simulink model "softdrone_pid"  (R2023b)
settings: Solver=FixedStepAuto  StartTime=0.0  StopTime=Inf  FixedStep=0.001  RelTol=1e-3
values from neighbouring files (symbols this model uses):
  DEG2RAD = 0.0174533    [Init_control450.m]
  K_ROLL_AngleRate = 1.0    (= 1)    [Init_control450.m]
  Kd_PITCH_AngleRate = 0.003    [Init_control450.m]
  Kd_ROLL_AngleRate = 0.003    [Init_control450.m]
  Kd_YAW_AngleRate = 0.01    [Init_control450.m]
  Ki_PITCH_AngleRate = 0.002    [Init_control450.m]
  Ki_ROLL_AngleRate = 0.002    [Init_control450.m]
  Ki_YAW_AngleRate = 0.0    (= 0)    [Init_control450.m]
  Kp_ANGLE = 1.0    (= 1)    [Init_control450.m]
  Kp_ROLL_AngleRate = 0.122    [Init_control450.m]
  Kp_YAW_AngleRate = 1.0    (= 1)    [Init_control450.m]
  MAX_CONTROL_ANGLE_PITCH = 35    [Init_control450.m]
  MAX_CONTROL_ANGLE_RATE_PITCH = 350    [Init_control450.m]
  MAX_CONTROL_ANGLE_RATE_ROLL = 350    [Init_control450.m]
  MAX_CONTROL_ANGLE_RATE_YAW = 250    [Init_control450.m]
  MAX_CONTROL_ANGLE_ROLL = 35    [Init_control450.m]
  Saturation_I_RP_Max = 0.3    [Init_control450.m]
  Saturation_I_RP_Min = -0.3    [Init_control450.m]
  THR_HOVER = 0.609    [Init_control450.m]
  TIME_Constant = 0.1    [Init_control450.m]
undefined symbols (not defined in the file or in its folder): DiscIntNeverNeededParam
libraries: ros2lib x7, simulink x3
settings Model: SimulationMode=external  Creator=hang  LastModifiedBy=root
settings SolverCC: AlgebraicLoopSolver=TrustRegion  AutoInsertRateTranBlk=on  DecoupledContinuousIntegration=on  MinimalZcImpactIntegration=on
settings DataIOCC: ReturnWorkspaceOutputs=off
settings OptimizationCC: EnhancedBackFolding=on  PassReuseOutputArgsAs=Individual arguments  ZeroExternalMemoryAtStartup=off  ZeroInternalMemoryAtStartup=off  MaxStackSize=64  OptimizeBlockOrder=speed  DifferentSizesBufferReuse=on  OptimizationCustomize=off  EfficientTunableParamExpr=on
settings DebuggingCC: ParameterTunabilityLossMsg=error  UnconnectedInputMsg=warning  UnconnectedOutputMsg=warning  UnconnectedLineMsg=warning  ArithmeticOperatorsInVariantConditions=warning
settings HardwareCC: ProdBitPerLong=64  ProdHWDeviceType=AMD->x86-64 (Linux 64)
settings ModelReferenceCC: EnableRefExpFcnMdlSchedulingChecks=on
settings SFSimCC: SimUseLocalCustomCode=off  MATLABDynamicMemAlloc=off  CustomCodeUndefinedFunction=UseInterfaceOnly
settings RTWCC: Description=Embedded Coder  SystemTargetFile=ert.tlc  HardwareBoard=Robot Operating System 2 (ROS 2)  TLCOptions="-aInlineSetEventsForThisBaseRateFcn=TLC_FALSE -aSuppressMultiTaskScheduler=TLC_FALSE  -aRateBasedStepFcn=0"  GenCodeOnly=on  TemplateMakefile=ert_default_tmf  RTWUseLocalCustomCode=off  Toolchain=Colcon Tools  TargetLang=C++  DLArmComputeVersion=19.05
settings CodeAppCC: ForceParamTrailComments=on  IgnoreCustomStorageClasses=off  MaxIdLength=95  OperatorAnnotations=on  SimulinkDataObjDesc=on  SFDataObjDesc=on  InsertBlockDesc=on
settings ERTTargetCC: ExtMode=on  ExtModeMexArgs='127.0.0.1' 0 17725  RootIOFormat=Structure reference

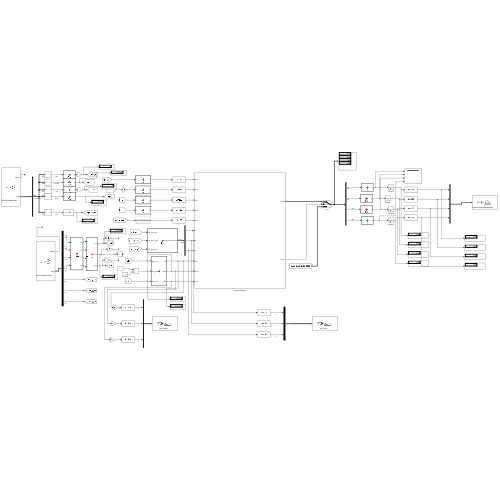
[thumbnail: Simulink's stored preview of the top-level diagram]
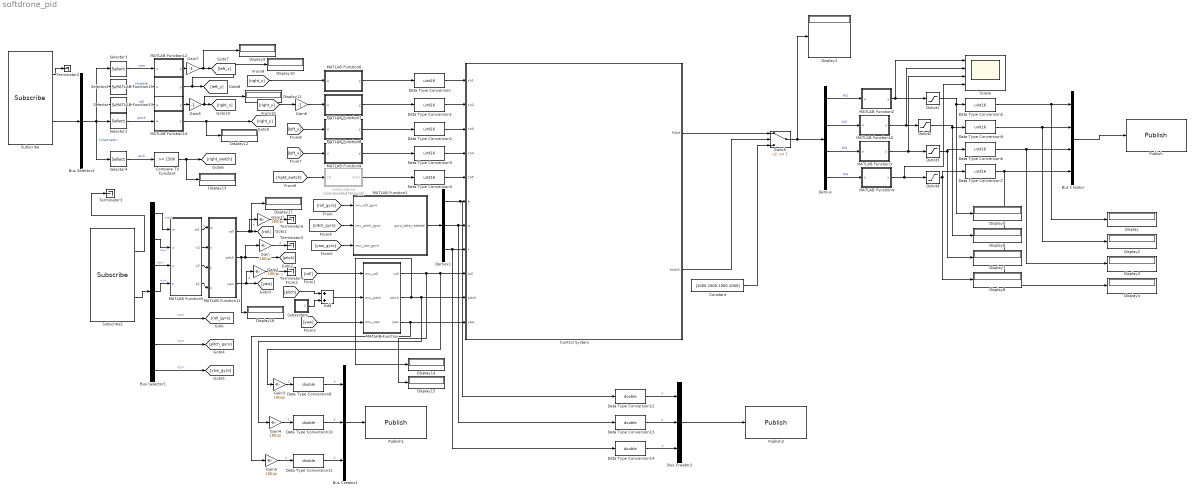
== system softdrone_pid ==
  Add : Sum
  Bus Creator : BusCreator  Inputs=4  OutDataTypeStr=Bus: SL_Bus_custom_msgs_WriteOnBoardPWM  NonVirtualBus=on
      settings: InheritFromInputs=off
  Bus Creator1 : BusCreator  Inputs=3  OutDataTypeStr=Bus: SL_Bus_geometry_msgs_Vector3  NonVirtualBus=on
  Bus Creator2 : BusCreator  Inputs=3  OutDataTypeStr=Bus: SL_Bus_geometry_msgs_Vector3  NonVirtualBus=on
  Bus Selector1 : BusSelector  OutputSignals=orientation.w,orientation.x,orientation.y,orientation.z,angular_velocity.x,angular_velocity.y,angular_velocity.z
  Bus Selector2 : BusSelector  OutputSignals=channels
  Compare To Constant : simulink/Logic and Bit Operations/Compare To Constant  relop=>=  const=1500  OutDataTypeStr=boolean
  Constant : Constant  Value=[1000,1000,1000,1000]
  Control System : Subsystem
  Data Type Conversion{,1..7,9} (9 alike) : DataTypeConversion  OutDataTypeStr=uint16  SaturateOnIntegerOverflow=off  RndMeth=Floor
  Data Type Conversion{8,10..14} (6 alike) : DataTypeConversion  OutDataTypeStr=double  SaturateOnIntegerOverflow=off  RndMeth=Floor
  Demux : Demux
  Demux1 : Demux  Outputs=3
  Display{,1..17} (18 alike) : Display
  Dshot{1..4} (4 alike) : Saturate  UpperLimit=2000  LowerLimit=1000
  Gain{,1..5} (6 alike) : Gain  Gain=180/pi
  Gain6 : Gain  Gain=-1
  Gain7 : Gain  Gain=-1
  Gain8 : Gain  Gain=-1
  MATLAB Function : MATLAB Function  TreatAsAtomicUnit=on
  MATLAB Function1 : MATLAB Function  TreatAsAtomicUnit=on
  MATLAB Function10 : MATLAB Function  TreatAsAtomicUnit=on
  MATLAB Function11 : MATLAB Function  TreatAsAtomicUnit=on
  MATLAB Function12 : MATLAB Function  TreatAsAtomicUnit=on
  MATLAB Function13 : MATLAB Function  TreatAsAtomicUnit=on
  MATLAB Function14 : MATLAB Function  TreatAsAtomicUnit=on
  MATLAB Function15 : MATLAB Function  TreatAsAtomicUnit=on
  MATLAB Function2 : MATLAB Function  TreatAsAtomicUnit=on
  MATLAB Function3 : MATLAB Function  TreatAsAtomicUnit=on
  MATLAB Function4 : MATLAB Function  TreatAsAtomicUnit=on
  MATLAB Function5 : MATLAB Function  TreatAsAtomicUnit=on
  MATLAB Function6 : MATLAB Function  TreatAsAtomicUnit=on
  MATLAB Function7 : MATLAB Function  TreatAsAtomicUnit=on
  MATLAB Function8 : MATLAB Function  TreatAsAtomicUnit=on
  MATLAB Function9 : MATLAB Function  TreatAsAtomicUnit=on
  Publish : ros2lib/Publish  topicSource=Select from ROS network  topic=/ecat/sn1966143/app3/write  messageType=custom_msgs/WriteOnBoardPWM  QOSHistory=Keep last  QOSDepth=1  QOSReliability=Best effort  QOSDurability=Volatile
  Publish1 : ros2lib/Publish  topicSource=Specify your own  topic=/imu_angle  messageType=geometry_msgs/Vector3  QOSHistory=Keep last  QOSDepth=1  QOSReliability=Reliable  QOSDurability=Volatile
  Publish2 : ros2lib/Publish  topicSource=Specify your own  topic=/imu_gyro  messageType=geometry_msgs/Vector3  QOSHistory=Keep all  QOSDepth=1  QOSReliability=Reliable  QOSDurability=Volatile
  Scope : Scope  NumInputPorts=4
  Selector : Selector  InputPortWidth=128  IndexOptions=Index vector (dialog)  Indices=1  OutputSizes=1
  Selector1 : Selector  InputPortWidth=128  IndexOptions=Index vector (dialog)  Indices=2  OutputSizes=1
  Selector2 : Selector  InputPortWidth=128  IndexOptions=Index vector (dialog)  Indices=3  OutputSizes=1
  Selector3 : Selector  InputPortWidth=128  IndexOptions=Index vector (dialog)  Indices=4  OutputSizes=1
  Selector4 : Selector  InputPortWidth=128  IndexOptions=Index vector (dialog)  Indices=5  OutputSizes=1
  Subscribe : ros2lib/Subscribe  topicSource=Select from ROS network  topic=/ecat/sn1966143/app1/read  messageType=custom_msgs/ReadSBUSRC  sampleTime=-1  QOSHistory=Keep last  QOSDepth=1  QOSReliability=Best effort  QOSDurability=Volatile
  Subscribe1 : ros2lib/Subscribe  topicSource=Select from ROS network  topic=/ecat/sn1966143/app2/read  messageType=sensor_msgs/Imu  sampleTime=-1  QOSHistory=Keep last  QOSDepth=1  QOSReliability=Best effort  QOSDurability=Volatile
  Subsystem : Subsystem
  Subsystem4 : Subsystem  Commented=through
  Switch : Switch  Threshold=1  SaturateOnIntegerOverflow=off  InputSameDT=off
  Terminator{2..6} (5 alike) : Terminator
  wires:
  Demux1/3 -> Data Type Conversion14/1, Control System/8(r)
  Demux1/1 -> Data Type Conversion12/1, Control System/6(p)
  MATLAB Function/2(pitch) -> Display14/1, Gain4/1, Control System/10(pitch)
  Demux1/2 -> Data Type Conversion13/1, Control System/7(q)
  Demux/4 -> MATLAB Function4/1(u)  "M4"
  Demux/3 -> MATLAB Function3/1(u)  "M3"
  Control System/1(PWM) -> Switch/1
  MATLAB Function1/1(gyro_data_rotated) -> Demux1/1
  MATLAB Function6/1(y) -> Data Type Conversion/1
  MATLAB Function9/1(y) -> Data Type Conversion3/1
  MATLAB Function8/1(y) -> Data Type Conversion2/1
  MATLAB Function7/1(y) -> Data Type Conversion1/1
  Subsystem4/1(Out1) -> Data Type Conversion4/1
  Control System/2(switch) -> Switch/2
  Data Type Conversion/1 -> Control System/1(ch1)
  Data Type Conversion1/1 -> Control System/2(ch2)
  Data Type Conversion2/1 -> Control System/3(ch3)
  Data Type Conversion3/1 -> Control System/4(ch4)
  Data Type Conversion4/1 -> Control System/5(ch5)
  Constant/1 -> Switch/3
  Switch/1 -> Display1/1, Demux/1
  Selector3/1 -> MATLAB Function12/1(u)  "yaw"
  Subscribe1/2 -> Bus Selector1/1
  Bus Creator/1 -> Publish/1
  MATLAB Function2/1(y) -> Scope/1, Dshot1/1
  MATLAB Function10/1(y) -> Scope/2, Dshot2/1
  MATLAB Function3/1(y) -> Scope/3, Dshot3/1
  MATLAB Function4/1(y) -> Scope/4, Dshot4/1
  Data Type Conversion5/1 -> Bus Creator/1, Display/1
  Data Type Conversion9/1 -> Bus Creator/2, Display2/1
  Data Type Conversion6/1 -> Bus Creator/3, Display3/1
  Data Type Conversion7/1 -> Bus Creator/4, Display4/1
  [roll_gyro] -> MATLAB Function1/1(imu_roll_gyro)
  [yaw] -> MATLAB Function/3(imu_yaw)
  [pitch_gyro] -> MATLAB Function1/2(imu_pitch_gyro)
  [yaw_gyro] -> MATLAB Function1/3(imu_yaw_gyro)
  [right_switch] -> Subsystem4/1(In1)
  [left_x] -> MATLAB Function9/1(u)
  [left_y] -> MATLAB Function8/1(u)
  Bus Selector1/7 -> [yaw_gyro]  "<z>"
  Bus Selector1/1 -> MATLAB Function5/1(w)  "<w>"
  Bus Selector1/4 -> MATLAB Function5/4(z)  "<z>"
  Subscribe/1 -> Terminator2/1
  Subscribe1/1 -> Terminator3/1
  Bus Selector1/2 -> MATLAB Function5/2(x)  "<x>"
  Bus Selector1/3 -> MATLAB Function5/3(y)  "<y>"
  MATLAB Function5/1(w2) -> MATLAB Function11/1(w)  "y"
  MATLAB Function5/2(x2) -> MATLAB Function11/2(x)
  MATLAB Function5/3(y2) -> MATLAB Function11/3(y)
  MATLAB Function5/4(z2) -> MATLAB Function11/4(z)
  Demux/1 -> MATLAB Function2/1(u)  "M1"
  Demux/2 -> MATLAB Function10/1(u)  "M2"
  MATLAB Function11/2(pitch) -> [pitch], Gain/1, Display16/1
  MATLAB Function11/3(yaw) -> Gain2/1, [yaw]  "z"
  MATLAB Function11/1(roll) -> Gain1/1, Display17/1, [roll]  "x"
  Bus Creator1/1 -> Publish1/1
  Data Type Conversion8/1 -> Bus Creator1/1  "x"
  Data Type Conversion10/1 -> Bus Creator1/2  "y"
  Data Type Conversion11/1 -> Bus Creator1/3  "z"
  Bus Creator2/1 -> Publish2/1
  Data Type Conversion12/1 -> Bus Creator2/1  "x"
  Data Type Conversion14/1 -> Bus Creator2/3  "z"
  Data Type Conversion13/1 -> Bus Creator2/2  "y"
  Bus Selector1/5 -> [roll_gyro]  "<x>"
  Bus Selector1/6 -> [pitch_gyro]  "<y>"
  Dshot2/1 -> Display6/1, Data Type Conversion9/1
  Dshot1/1 -> Display5/1, Data Type Conversion5/1
  Dshot3/1 -> Data Type Conversion6/1, Display7/1
  Dshot4/1 -> Display8/1, Data Type Conversion7/1
  MATLAB Function/3(yaw) -> Control System/11(yaw), Gain5/1
  Gain3/1 -> Data Type Conversion8/1  "z"
  Gain4/1 -> Data Type Conversion10/1  "z"
  Gain5/1 -> Data Type Conversion11/1  "z"
  Gain2/1 -> Terminator4/1  "z"
  Gain/1 -> Terminator5/1  "y"
  Gain1/1 -> Terminator6/1  "x"
  [right_y] -> Gain6/1
  [right_x] -> MATLAB Function6/1(u)
  Gain6/1 -> MATLAB Function7/1(u)
  Subscribe/2 -> Bus Selector2/1
  Bus Selector2/1 -> Selector4/1, Selector1/1, Selector3/1, Selector2/1, Selector/1  "<channels>"
  Selector/1 -> MATLAB Function13/1(u)  "roll"
  Selector1/1 -> MATLAB Function14/1(u)  "pitch"
  Selector2/1 -> MATLAB Function15/1(u)  "throttle"
  Selector4/1 -> Compare To Constant/1  "arm"
  MATLAB Function14/1(y) -> Display12/1, [right_y]
  MATLAB Function15/1(y) -> Display10/1, [left_y]
  Compare To Constant/1 -> Display13/1, [right_switch]
  MATLAB Function12/1(y) -> Gain7/1
  Gain7/1 -> Display9/1, [left_x]
  MATLAB Function13/1(y) -> Gain8/1
  Gain8/1 -> Display11/1, [right_x]
  MATLAB Function/1(roll) -> Display15/1, Gain3/1, Control System/9(roll)
  [roll] -> MATLAB Function/1(imu_roll)
  [pitch] -> Add/1
  Add/1 -> MATLAB Function/2(imu_pitch)
  Subsystem/1(Out1) -> Add/2

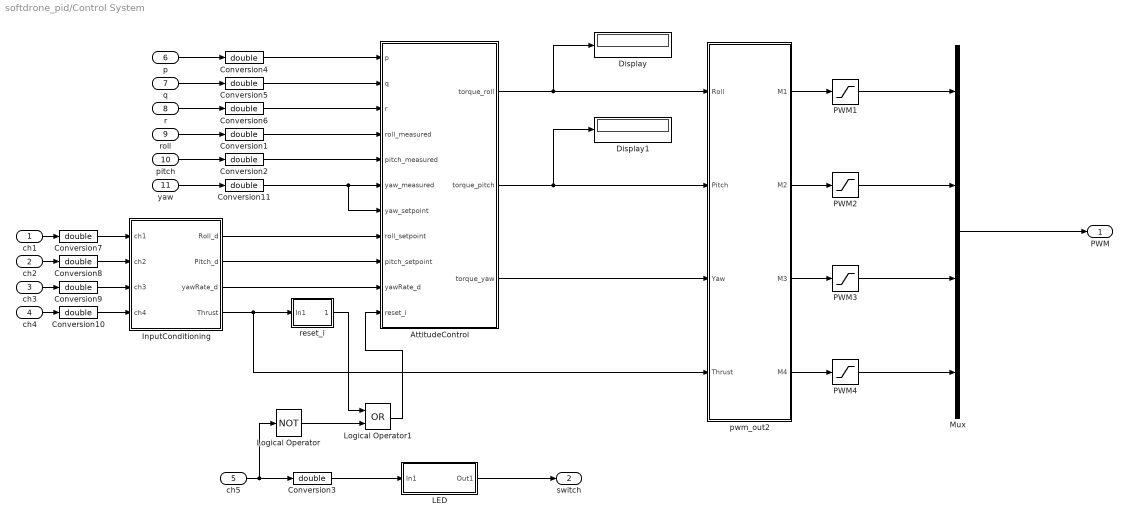
== system softdrone_pid/Control System ==
  ch1 : Inport  OutDataTypeStr=uint16  PortDimensions=1
  ch2 : Inport  Port=2  OutDataTypeStr=uint16  PortDimensions=1
  ch3 : Inport  Port=3  OutDataTypeStr=uint16  PortDimensions=1
  ch4 : Inport  Port=4  OutDataTypeStr=uint16  PortDimensions=1
  ch5 : Inport  Port=5  OutDataTypeStr=uint16  PortDimensions=1  Interpolate=off
  p : Inport  Port=6  PortDimensions=1
  q : Inport  Port=7  PortDimensions=1
  r : Inport  Port=8  PortDimensions=1
  roll : Inport  Port=9  PortDimensions=1
  pitch : Inport  Port=10  PortDimensions=1
  yaw : Inport  Port=11  PortDimensions=1
  AttitudeControl : Subsystem
  Conversion{1..11} (11 alike) : DataTypeConversion  OutDataTypeStr=double  SaturateOnIntegerOverflow=off  RndMeth=Floor
  Display : Display
  Display1 : Display
  InputConditioning : Subsystem
  "LED " : Subsystem
  Logical Operator : Logic  Operator=NOT  AllPortsSameDT=off  OutDataTypeStr=boolean
  Logical Operator1 : Logic  Operator=OR  AllPortsSameDT=off  OutDataTypeStr=boolean
  Mux : Mux
  PWM{1..4} (4 alike) : Saturate  UpperLimit=2000  LowerLimit=1200
  pwm_out2 : MATLAB Function  SystemSampleTime=0.004
  reset_i : Subsystem
  PWM : Outport  VectorParamsAs1DForOutWhenUnconnected=off
  switch : Outport  Port=2  PortDimensions=1  VectorParamsAs1DForOutWhenUnconnected=off
  wires:
  AttitudeControl/2(torque_pitch) -> Display1/1, pwm_out2/2(Pitch)
  AttitudeControl/3(torque_yaw) -> pwm_out2/3(Yaw)
  reset_i/1(Out1) -> Logical Operator1/1
  p/1 -> Conversion4/1
  q/1 -> Conversion5/1
  r/1 -> Conversion6/1
  pitch/1 -> Conversion2/1
  roll/1 -> Conversion1/1
  "LED "/1(Out1) -> switch/1
  ch5/1 -> Logical Operator/1, Conversion3/1
  Conversion3/1 -> "LED "/1(In1)
  ch3/1 -> Conversion9/1
  ch4/1 -> Conversion10/1
  Conversion10/1 -> InputConditioning/4(ch4)
  Conversion9/1 -> InputConditioning/3(ch3)
  ch1/1 -> Conversion7/1
  ch2/1 -> Conversion8/1
  InputConditioning/3(yawRate_d) -> AttitudeControl/10(yawRate_d)
  InputConditioning/4(Thrust) -> pwm_out2/4(Thrust), reset_i/1(In1)
  Conversion7/1 -> InputConditioning/1("ch1 ")
  Conversion8/1 -> InputConditioning/2(ch2)
  yaw/1 -> Conversion11/1
  Conversion6/1 -> AttitudeControl/3(r)
  Conversion5/1 -> AttitudeControl/2(q)
  Conversion4/1 -> AttitudeControl/1(p)
  Conversion11/1 -> AttitudeControl/6(yaw_measured), AttitudeControl/7(yaw_setpoint)
  Conversion2/1 -> AttitudeControl/5(pitch_measured)
  Conversion1/1 -> AttitudeControl/4(roll_measured)
  InputConditioning/2(Pitch_d) -> AttitudeControl/9(pitch_setpoint)
  InputConditioning/1(Roll_d) -> AttitudeControl/8(roll_setpoint)
  AttitudeControl/1(torque_roll) -> Display/1, pwm_out2/1(Roll)
  pwm_out2/4(M4) -> PWM4/1
  pwm_out2/3(M3) -> PWM3/1
  pwm_out2/1(M1) -> PWM1/1
  pwm_out2/2(M2) -> PWM2/1
  Mux/1 -> PWM/1
  PWM1/1 -> Mux/1
  PWM2/1 -> Mux/2
  PWM3/1 -> Mux/3
  PWM4/1 -> Mux/4
  Logical Operator/1 -> Logical Operator1/2
  Logical Operator1/1 -> AttitudeControl/11(reset_i)

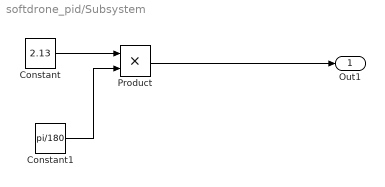
== system softdrone_pid/Subsystem ==
  Constant : Constant  Value=2.13
  Constant1 : Constant  Value=pi/180
  Product : Product
  Out1 : Outport
  wires:
  Constant/1 -> Product/1
  Constant1/1 -> Product/2
  Product/1 -> Out1/1

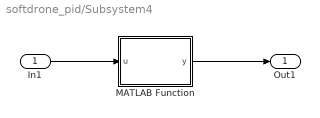
== system softdrone_pid/Subsystem4 ==
  In1 : Inport
  MATLAB Function : MATLAB Function  TreatAsAtomicUnit=on
  Out1 : Outport
  wires:
  In1/1 -> MATLAB Function/1(u)
  MATLAB Function/1(y) -> Out1/1

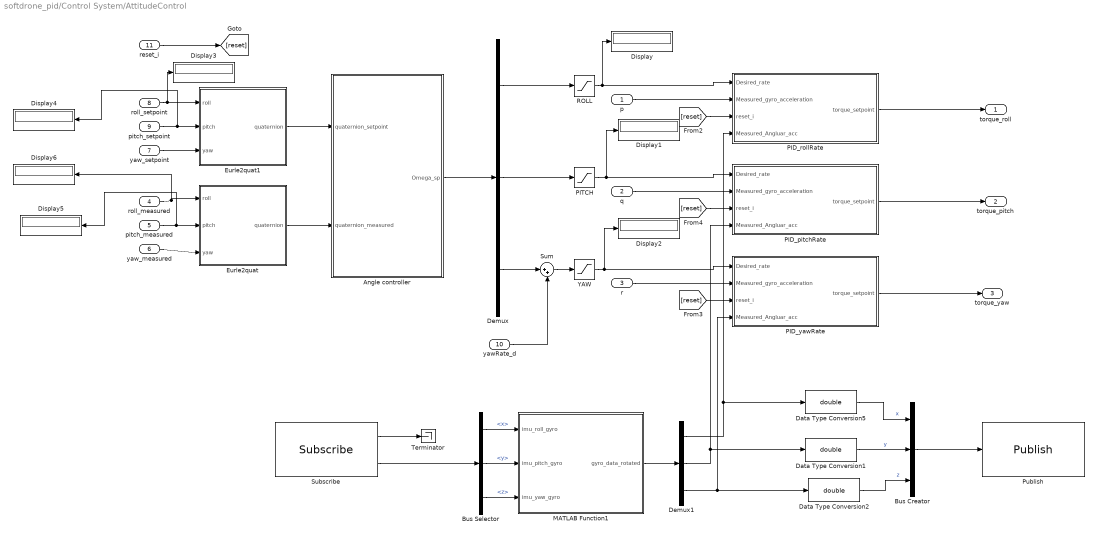
== system softdrone_pid/Control System/AttitudeControl ==
  p : Inport
  q : Inport  Port=2
  r : Inport  Port=3
  roll_measured : Inport  Port=4
  pitch_measured : Inport  Port=5
  yaw_measured : Inport  Port=6
  yaw_setpoint : Inport  Port=7
  roll_setpoint : Inport  Port=8
  pitch_setpoint : Inport  Port=9
  yawRate_d : Inport  Port=10
  reset_i : Inport  Port=11
  Angle controller : Subsystem
  Bus Creator : BusCreator  Inputs=3  OutDataTypeStr=Bus: SL_Bus_geometry_msgs_Vector3  NonVirtualBus=on
  Bus Selector : BusSelector  OutputSignals=x,y,z
  Data Type Conversion1 : DataTypeConversion  OutDataTypeStr=double  SaturateOnIntegerOverflow=off  RndMeth=Floor
  Data Type Conversion2 : DataTypeConversion  OutDataTypeStr=double  SaturateOnIntegerOverflow=off  RndMeth=Floor
  Data Type Conversion5 : DataTypeConversion  OutDataTypeStr=double  SaturateOnIntegerOverflow=off  RndMeth=Floor
  Demux : Demux  Outputs=3
  Demux1 : Demux  Outputs=3
  Display{,1..6} (7 alike) : Display
  Eurle2quat : MATLAB Function  TreatAsAtomicUnit=on
  Eurle2quat1 : MATLAB Function  TreatAsAtomicUnit=on
  MATLAB Function1 : MATLAB Function  TreatAsAtomicUnit=on
  PID_pitchRate : Subsystem
  PID_rollRate : Subsystem
  PID_yawRate : Subsystem
  PITCH : Saturate  UpperLimit=MAX_CONTROL_ANGLE_RATE_PITCH  LowerLimit=-MAX_CONTROL_ANGLE_RATE_PITCH
  Publish : ros2lib/Publish  topicSource=Specify your own  topic=/gyro_rotated  messageType=geometry_msgs/Vector3  QOSHistory=Keep last  QOSDepth=1  QOSReliability=Best effort  QOSDurability=Volatile
  ROLL : Saturate  UpperLimit=MAX_CONTROL_ANGLE_RATE_ROLL  LowerLimit=-MAX_CONTROL_ANGLE_RATE_ROLL
  Subscribe : ros2lib/Subscribe  topicSource=Select from ROS network  topic=/filtered_angular_acceleration  messageType=geometry_msgs/Vector3  sampleTime=-1  QOSHistory=Keep last  QOSDepth=1  QOSReliability=Reliable  QOSDurability=Volatile
  Sum : Sum  Inputs=|++
  Terminator : Terminator
  YAW : Saturate  UpperLimit=MAX_CONTROL_ANGLE_RATE_YAW  LowerLimit=-MAX_CONTROL_ANGLE_RATE_YAW
  torque_roll : Outport  VectorParamsAs1DForOutWhenUnconnected=off
  torque_pitch : Outport  Port=2  VectorParamsAs1DForOutWhenUnconnected=off
  torque_yaw : Outport  Port=3  VectorParamsAs1DForOutWhenUnconnected=off
  wires:
  p/1 -> PID_rollRate/2(Measured_gyro_acceleration)
  reset_i/1 -> [reset]
  [reset] -> PID_rollRate/3(reset_i)
  PID_rollRate/1(torque_setpoint) -> torque_roll/1
  [reset] -> PID_pitchRate/3(reset_i)
  PID_pitchRate/1(torque_setpoint) -> torque_pitch/1
  q/1 -> PID_pitchRate/2(Measured_gyro_acceleration)
  [reset] -> PID_yawRate/3(reset_i)
  PID_yawRate/1(torque_setpoint) -> torque_yaw/1
  r/1 -> PID_yawRate/2(Measured_gyro_acceleration)
  Eurle2quat/1(quaternion) -> Angle controller/2(quaternion_measured)
  roll_measured/1 -> Display6/1, Eurle2quat/1(roll)
  pitch_measured/1 -> Display5/1, Eurle2quat/2(pitch)
  yaw_measured/1 -> Eurle2quat/3(yaw)
  Eurle2quat1/1(quaternion) -> Angle controller/1(quaternion_setpoint)
  pitch_setpoint/1 -> Display4/1, Eurle2quat1/2(pitch)
  roll_setpoint/1 -> Display3/1, Eurle2quat1/1(roll)
  yaw_setpoint/1 -> Eurle2quat1/3(yaw)
  Demux/1 -> ROLL/1
  Demux/2 -> PITCH/1
  Angle controller/1(Omega_sp) -> Demux/1
  Demux/3 -> Sum/1
  Sum/1 -> YAW/1
  yawRate_d/1 -> Sum/2
  ROLL/1 -> Display/1, PID_rollRate/1(Desired_rate)
  PITCH/1 -> Display1/1, PID_pitchRate/1(Desired_rate)
  YAW/1 -> Display2/1, PID_yawRate/1(Desired_rate)
  Subscribe/1 -> Terminator/1
  Subscribe/2 -> Bus Selector/1
  Bus Selector/1 -> MATLAB Function1/1(imu_roll_gyro)  "<x>"
  Bus Selector/2 -> MATLAB Function1/2(imu_pitch_gyro)  "<y>"
  Bus Selector/3 -> MATLAB Function1/3(imu_yaw_gyro)  "<z>"
  MATLAB Function1/1(gyro_data_rotated) -> Demux1/1
  Demux1/1 -> Data Type Conversion5/1, PID_rollRate/4(Measured_Angluar_acc)
  Demux1/3 -> Data Type Conversion2/1, PID_yawRate/4(Measured_Angluar_acc)
  Demux1/2 -> Data Type Conversion1/1, PID_pitchRate/4(Measured_Angluar_acc)
  Data Type Conversion5/1 -> Bus Creator/1  "x"
  Data Type Conversion1/1 -> Bus Creator/2  "y"
  Data Type Conversion2/1 -> Bus Creator/3  "z"
  Bus Creator/1 -> Publish/1

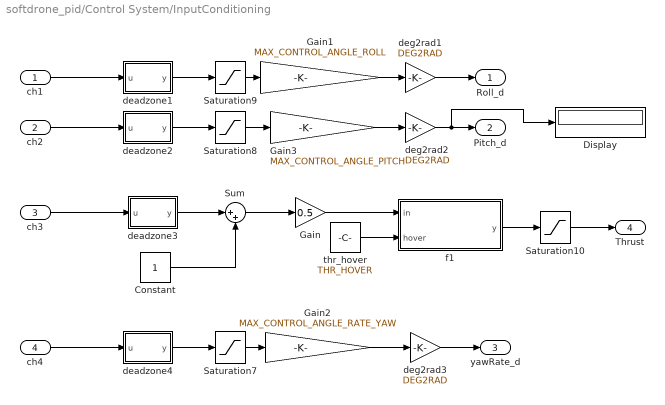
== system softdrone_pid/Control System/InputConditioning ==
  "ch1 " : Inport
  ch2 : Inport  Port=2
  ch3 : Inport  Port=3
  ch4 : Inport  Port=4
  Constant : Constant
  Display : Display
  Gain : Gain  Gain=0.5
  Gain1 : Gain  Gain=MAX_CONTROL_ANGLE_ROLL  OutDataTypeStr=Inherit: Inherit via back propagation
  Gain2 : Gain  Gain=MAX_CONTROL_ANGLE_RATE_YAW
  Gain3 : Gain  Gain=MAX_CONTROL_ANGLE_PITCH  OutDataTypeStr=Inherit: Inherit via back propagation
  Saturation10 : Saturate  UpperLimit=1  LowerLimit=0
  Saturation7 : Saturate  UpperLimit=1  LowerLimit=-1
  Saturation8 : Saturate  UpperLimit=1  LowerLimit=-1
  Saturation9 : Saturate  UpperLimit=1  LowerLimit=-1
  Sum : Sum  Inputs=|++
  deadzone1 : MATLAB Function  TreatAsAtomicUnit=on
  deadzone2 : MATLAB Function  TreatAsAtomicUnit=on
  deadzone3 : MATLAB Function  TreatAsAtomicUnit=on
  deadzone4 : MATLAB Function  TreatAsAtomicUnit=on
  deg2rad1 : Gain  Gain=DEG2RAD
  deg2rad2 : Gain  Gain=DEG2RAD
  deg2rad3 : Gain  Gain=DEG2RAD
  f1 : MATLAB Function  TreatAsAtomicUnit=on
  "thr_hover " : Constant  Value=THR_HOVER
  Roll_d : Outport  VectorParamsAs1DForOutWhenUnconnected=off
  Pitch_d : Outport  Port=2  VectorParamsAs1DForOutWhenUnconnected=off
  yawRate_d : Outport  Port=3  VectorParamsAs1DForOutWhenUnconnected=off
  Thrust : Outport  Port=4  VectorParamsAs1DForOutWhenUnconnected=off
  wires:
  deadzone3/1(y) -> Sum/1
  ch3/1 -> deadzone3/1(u)
  deadzone2/1(y) -> Saturation8/1
  Saturation10/1 -> Thrust/1
  deadzone1/1(y) -> Saturation9/1
  "ch1 "/1 -> deadzone1/1(u)
  ch2/1 -> deadzone2/1(u)
  Saturation9/1 -> Gain1/1
  Saturation8/1 -> Gain3/1
  Gain3/1 -> deg2rad2/1
  Constant/1 -> Sum/2
  Sum/1 -> Gain/1
  Gain1/1 -> deg2rad1/1
  deg2rad1/1 -> Roll_d/1
  deg2rad2/1 -> Display/1, Pitch_d/1
  Saturation7/1 -> Gain2/1
  deadzone4/1(y) -> Saturation7/1
  ch4/1 -> deadzone4/1(u)
  Gain2/1 -> deg2rad3/1
  deg2rad3/1 -> yawRate_d/1
  "thr_hover "/1 -> f1/2(hover)
  Gain/1 -> f1/1(in)
  f1/1(y) -> Saturation10/1

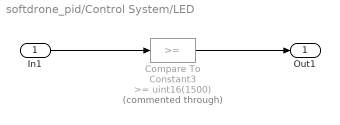
== system softdrone_pid/Control System/LED  ==
  In1 : Inport
  Compare To Constant3 : simulink/Logic and Bit Operations/Compare To Constant  Commented=through  relop=>=  const=uint16(1500)  OutDataTypeStr=boolean
  Out1 : Outport  VectorParamsAs1DForOutWhenUnconnected=off
  wires:
  Compare To Constant3/1 -> Out1/1
  In1/1 -> Compare To Constant3/1

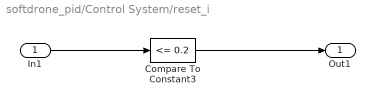
== system softdrone_pid/Control System/reset_i ==
  In1 : Inport
  Compare To Constant3 : simulink/Logic and Bit Operations/Compare To Constant  relop=<=  const=0.2  OutDataTypeStr=boolean
  Out1 : Outport  VectorParamsAs1DForOutWhenUnconnected=off
  wires:
  In1/1 -> Compare To Constant3/1
  Compare To Constant3/1 -> Out1/1

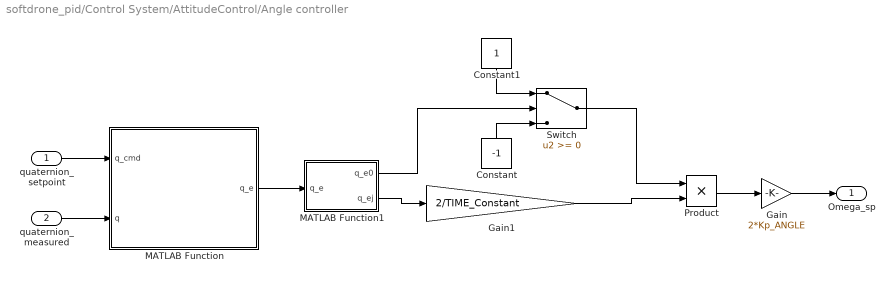
== system softdrone_pid/Control System/AttitudeControl/Angle controller ==
  quaternion_setpoint : Inport
  quaternion_measured : Inport  Port=2
  Constant : Constant  Value=-1
  Constant1 : Constant
  Gain : Gain  Gain=2*Kp_ANGLE
  Gain1 : Gain  Gain=2/TIME_Constant
  MATLAB Function : MATLAB Function  TreatAsAtomicUnit=on
  MATLAB Function1 : MATLAB Function  TreatAsAtomicUnit=on
  Product : Product
  Switch : Switch  SaturateOnIntegerOverflow=off  InputSameDT=off
  Omega_sp : Outport
  wires:
  quaternion_setpoint/1 -> MATLAB Function/1(q_cmd)
  quaternion_measured/1 -> MATLAB Function/2(q)
  Gain/1 -> Omega_sp/1
  Product/1 -> Gain/1
  MATLAB Function/1(q_e) -> MATLAB Function1/1(q_e)
  Gain1/1 -> Product/2
  MATLAB Function1/2(q_ej) -> Gain1/1
  MATLAB Function1/1(q_e0) -> Switch/2
  Switch/1 -> Product/1
  Constant/1 -> Switch/3
  Constant1/1 -> Switch/1

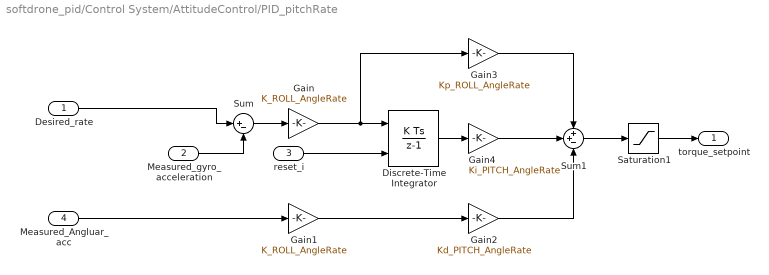
== system softdrone_pid/Control System/AttitudeControl/PID_pitchRate ==
  Desired_rate : Inport
  Measured_gyro_acceleration : Inport  Port=2
  reset_i : Inport  Port=3
  Measured_Angluar_acc : Inport  Port=4
  Discrete-Time Integrator : DiscreteIntegrator  ExternalReset=level  SampleTime=-1  LimitOutput=on  UpperSaturationLimit=Saturation_I_RP_Max  LowerSaturationLimit=Saturation_I_RP_Min  ICPrevOutput=DiscIntNeverNeededParam  ICPrevScaledInput=DiscIntNeverNeededParam
  Gain : Gain  Gain=K_ROLL_AngleRate
  Gain1 : Gain  Gain=K_ROLL_AngleRate
  Gain2 : Gain  Gain=Kd_PITCH_AngleRate
  Gain3 : Gain  Gain=Kp_ROLL_AngleRate
  Gain4 : Gain  Gain=Ki_PITCH_AngleRate
  Saturation1 : Saturate  UpperLimit=1  LowerLimit=-1
  Sum : Sum  Inputs=|+-
  Sum1 : Sum  Inputs=++-
  torque_setpoint : Outport
  wires:
  Gain2/1 -> Sum1/3
  Gain4/1 -> Sum1/2
  Gain3/1 -> Sum1/1
  Gain/1 -> Discrete-Time Integrator/1, Gain3/1
  Sum1/1 -> Saturation1/1
  Saturation1/1 -> torque_setpoint/1
  Discrete-Time Integrator/1 -> Gain4/1
  reset_i/1 -> Discrete-Time Integrator/2
  Gain1/1 -> Gain2/1
  Desired_rate/1 -> Sum/1
  Sum/1 -> Gain/1
  Measured_gyro_acceleration/1 -> Sum/2
  Measured_Angluar_acc/1 -> Gain1/1

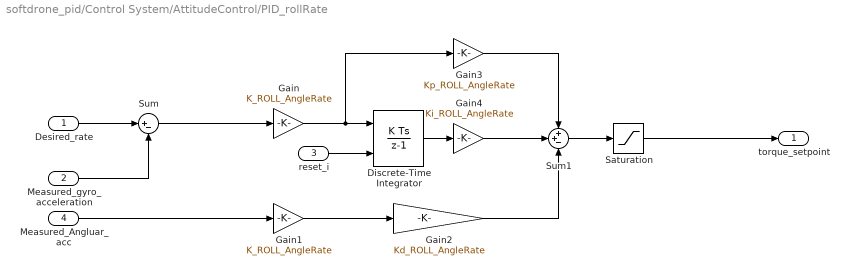
== system softdrone_pid/Control System/AttitudeControl/PID_rollRate ==
  Desired_rate : Inport
  Measured_gyro_acceleration : Inport  Port=2
  reset_i : Inport  Port=3
  Measured_Angluar_acc : Inport  Port=4
  Discrete-Time Integrator : DiscreteIntegrator  ExternalReset=level  SampleTime=-1  LimitOutput=on  UpperSaturationLimit=Saturation_I_RP_Max  LowerSaturationLimit=Saturation_I_RP_Min  ICPrevOutput=DiscIntNeverNeededParam  ICPrevScaledInput=DiscIntNeverNeededParam
  Gain : Gain  Gain=K_ROLL_AngleRate
  Gain1 : Gain  Gain=K_ROLL_AngleRate
  Gain2 : Gain  Gain=Kd_ROLL_AngleRate
  Gain3 : Gain  Gain=Kp_ROLL_AngleRate
  Gain4 : Gain  Gain=Ki_ROLL_AngleRate
  Saturation : Saturate  UpperLimit=1  LowerLimit=-1
  Sum : Sum  Inputs=|+-
  Sum1 : Sum  Inputs=++-
  torque_setpoint : Outport
  wires:
  Gain2/1 -> Sum1/3
  Gain4/1 -> Sum1/2
  Gain3/1 -> Sum1/1
  Gain/1 -> Discrete-Time Integrator/1, Gain3/1
  Sum1/1 -> Saturation/1
  Discrete-Time Integrator/1 -> Gain4/1
  reset_i/1 -> Discrete-Time Integrator/2
  Gain1/1 -> Gain2/1
  Desired_rate/1 -> Sum/1
  Measured_gyro_acceleration/1 -> Sum/2
  Sum/1 -> Gain/1
  Measured_Angluar_acc/1 -> Gain1/1
  Saturation/1 -> torque_setpoint/1

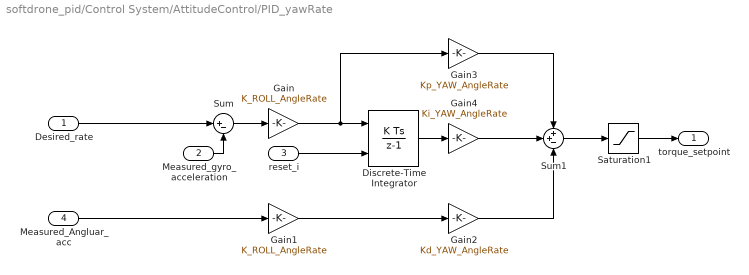
== system softdrone_pid/Control System/AttitudeControl/PID_yawRate ==
  Desired_rate : Inport
  Measured_gyro_acceleration : Inport  Port=2
  reset_i : Inport  Port=3
  Measured_Angluar_acc : Inport  Port=4
  Discrete-Time Integrator : DiscreteIntegrator  ExternalReset=level  SampleTime=-1  LimitOutput=on  UpperSaturationLimit=Saturation_I_RP_Max  LowerSaturationLimit=Saturation_I_RP_Min  ICPrevOutput=DiscIntNeverNeededParam  ICPrevScaledInput=DiscIntNeverNeededParam
  Gain : Gain  Gain=K_ROLL_AngleRate
  Gain1 : Gain  Gain=K_ROLL_AngleRate
  Gain2 : Gain  Gain=Kd_YAW_AngleRate
  Gain3 : Gain  Gain=Kp_YAW_AngleRate
  Gain4 : Gain  Gain=Ki_YAW_AngleRate
  Saturation1 : Saturate  UpperLimit=1  LowerLimit=-1
  Sum : Sum  Inputs=|+-
  Sum1 : Sum  Inputs=++-
  torque_setpoint : Outport
  wires:
  Gain2/1 -> Sum1/3
  Gain4/1 -> Sum1/2
  Gain3/1 -> Sum1/1
  Gain/1 -> Discrete-Time Integrator/1, Gain3/1
  Sum1/1 -> Saturation1/1
  Saturation1/1 -> torque_setpoint/1
  Discrete-Time Integrator/1 -> Gain4/1
  reset_i/1 -> Discrete-Time Integrator/2
  Gain1/1 -> Gain2/1
  Desired_rate/1 -> Sum/1
  Sum/1 -> Gain/1
  Measured_gyro_acceleration/1 -> Sum/2
  Measured_Angluar_acc/1 -> Gain1/1

== matlab function softdrone_pid/MATLAB Function6 ==
  data: u input; y output
function y = fcn(u)
y = u*500+1500;

== matlab function softdrone_pid/MATLAB Function7 ==
  data: u input; y output
function y = fcn(u)
y = u*500+1500;

== matlab function softdrone_pid/Control System/pwm_out2 ==
  data: Roll input; M1 output; Pitch input; Yaw input; Thrust input; M2 output; M3 output; M4 output
function [M1, M2, M3, M4] = motor_mixer(Roll, Pitch, Yaw, Thrust)
%Function description:
%  Control allocation. The quadrotor type is X-configuration,
%  and the airframe is as follows:
%3↓   1↑
 %  \ /
 %  / \
 %2↑   4↓
%Input：
%  Roll, Pitch, Yaw: attitude controller output.
%  Thrust

idle_PWM = 1000;
scale = 1000;

M1 = (Thrust - Roll + Pitch + Yaw) * scale + idle_PWM;
M2 = (Thrust + Roll - Pitch + Yaw) * scale + idle_PWM;
M3 = (Thrust + Roll + Pitch - Yaw) * scale + idle_PWM;
M4 = (Thrust - Roll - Pitch - Yaw) * scale + idle_PWM;

== matlab function softdrone_pid/MATLAB Function8 ==
  data: u input; y output
function y = fcn(u)
y = u*500+1500;

== matlab function softdrone_pid/MATLAB Function9 ==
  data: u input; y output
function y = fcn(u)
y = u*500+1500;

== matlab function softdrone_pid/MATLAB Function10 ==
  data: u input; y output
function y = fcn(u)
% Onboard PWM output
% Input : PWM pulse width in us
% Output: uint16, limited to 1000~2000 us

u = double(u);

if u < 1000
    u = 1000;
elseif u > 2000
    u = 2000;
end

y = uint16(round(u));
end

== matlab function softdrone_pid/Control System/AttitudeControl/Eurle2quat1 ==
  data: roll input; quaternion output; pitch input; yaw input
function quaternion = fcn(roll, pitch, yaw)

eul = [yaw, pitch, roll];
quaternion = eul2quat(eul);

== matlab function softdrone_pid/Control System/AttitudeControl/Angle controller/MATLAB Function ==
  data: q_cmd input; q input; q_e output
function q_e = calculateErrorQuaternion(q_cmd, q)
    %#codegen
    % 计算当前姿态四元数的共轭（即逆）
    q_conj = [q(1), -q(2), -q(3), -q(4)];

    % 计算误差四元数 q_e = q_conj * q_cmd
    q_e = zeros(1, 4);
    q_e(1) = q_conj(1) * q_cmd(1) - q_conj(2) * q_cmd(2) - q_conj(3) * q_cmd(3) - q_conj(4) * q_cmd(4);
    q_e(2) = q_conj(1) * q_cmd(2) + q_conj(2) * q_cmd(1) + q_conj(3) * q_cmd(4) - q_conj(4) * q_cmd(3);
    q_e(3) = q_conj(1) * q_cmd(3) - q_conj(2) * q_cmd(4) + q_conj(3) * q_cmd(1) + q_conj(4) * q_cmd(2);
    q_e(4) = q_conj(1) * q_cmd(4) + q_conj(2) * q_cmd(3) - q_conj(3) * q_cmd(2) + q_conj(4) * q_cmd(1);
end


% function q_e = calculateErrorQuaternion(q, q_cmd)
%     %#codegen
%     % 计算当前姿态四元数的共轭（即逆）
%     q_conj = [q(1), -q(2), -q(3), -q(4)];
% 
%     % 计算误差四元数 q_e = q_conj * q_cmd
%     q_e = quaternionMultiply(q_conj, q_cmd);
% end
% 
% function q_product = quaternionMultiply(q1, q2)
%     % 四元数乘法
%     q_product = [
%         q1(1)*q2(1) - q1(2)*q2(2) - q1(3)*q2(3) - q1(4)*q2(4);
%         q1(1)*q2(2) + q1(2)*q2(1) + q1(3)*q2(4) - q1(4)*q2(3);
%         q1(1)*q2(3) - q1(2)*q2(4) + q1(3)*q2(1) + q1(4)*q2(2);
%         q1(1)*q2(4) + q1(2)*q2(3) - q1(3)*q2(2) + q1(4)*q2(1)
%     ];
% end

== matlab function softdrone_pid/Control System/AttitudeControl/Angle controller/MATLAB Function1 ==
  data: q_e input; q_e0 output; q_ej output
function [q_e0, q_ej]= fcn(q_e)

q_e0 = q_e(1);

q_ej = [q_e(2); q_e(3); q_e(4)];

== matlab function softdrone_pid/MATLAB Function5 ==
  data: w input; w2 output; x input; y input; z input; x2 output; y2 output; z2 output
function [w2, x2, y2, z2] = flip_x_axis_quat(w, x, y, z)
% 输入: 四元数(w, x, y, z), x向右y向前z向上
% 输出: 四元数(w2, x2, y2, z2), x反向(y/z不变)

% 四元数转旋转矩阵
R = quat2rotm([w x y z]);

% x轴取反变换矩阵
Mx = [-1 0 0;
       0 1 0;
       0 0 1];

% 应用镜像变换
R_flip = Mx * R * Mx;

% 旋转矩阵转回四元数
q2 = rotm2quat(R_flip);

% 保证四元数为标准形式
if q2(1)<0
    q2 = -q2;
end

% 输出
w2 = q2(1);
x2 = q2(2);
y2 = q2(3);
z2 = q2(4);
end

function R = quat2rotm(q)
% 四元数 -> 旋转矩阵，q=[w x y z]
w = q(1); x = q(2); y = q(3); z = q(4);
R = [1-2*(y^2+z^2), 2*(x*y-w*z),   2*(x*z+w*y);
     2*(x*y+w*z),   1-2*(x^2+z^2), 2*(y*z-w*x);
     2*(x*z-w*y),   2*(y*z+w*x),   1-2*(x^2+y^2)];
end

function q = rotm2quat(R)
% 旋转矩阵 -> 四元数，输出q=[w x y z]
tr = trace(R);
if tr > 0
    S = sqrt(tr+1.0)*2; % S=4*qw
    qw = 0.25*S;
    qx = (R(3,2)-R(2,3))/S;
    qy = (R(1,3)-R(3,1))/S;
    qz = (R(2,1)-R(1,2))/S;
elseif (R(1,1) > R(2,2)) && (R(1,1) > R(3,3))
    S = sqrt(1.0+R(1,1)-R(2,2)-R(3,3))*2;
    qw = (R(3,2)-R(2,3))/S;
    qx = 0.25*S;
    qy = (R(1,2)+R(2,1))/S;
    qz = (R(1,3)+R(3,1))/S;
elseif (R(2,2) > R(3,3))
    S = sqrt(1.0+R(2,2)-R(1,1)-R(3,3))*2;
    qw = (R(1,3)-R(3,1))/S;
    qx = (R(1,2)+R(2,1))/S;
    qy = 0.25*S;
    qz = (R(2,3)+R(3,2))/S;
else
    S = sqrt(1.0+R(3,3)-R(1,1)-R(2,2))*2;
    qw = (R(2,1)-R(1,2))/S;
    qx = (R(1,3)+R(3,1))/S;
    qy = (R(2,3)+R(3,2))/S;
    qz = 0.25*S;
end
q = [qw qx qy qz];
end

== matlab function softdrone_pid/Control System/InputConditioning/deadzone1 ==
  data: u input; y output
function y = fcn(u)
%Function description:
%  Control the range of the remote control input from RCMin to RCMax, and
%  set a dead zone with a dead zone size of ±deadZone. The output y is
%  normalized to 0~1.You can get the RC calibration parameters in QGC.
RCMin = 1100;
RCMax = 1900;
RCMid = (RCMin + RCMax)/2;
deadZoneRate = 0.05;
deadZone = deadZoneRate*(RCMax - RCMin);
k = 1/(RCMax - RCMid - deadZone);
% saturation
if(u < RCMin)
    u = RCMin;
elseif(u > RCMax)
    u = RCMax;
end
% dead zone and normalize
 if(u > RCMid + deadZone)
    y = (u-RCMid - deadZone)*k;
 elseif(u < RCMid - deadZone)
     y = (u - RCMid + deadZone)*k;
 else
     y = 0;
 end

 end

== matlab function softdrone_pid/MATLAB Function11 ==
  data: w input; roll output; x input; y input; z input; pitch output; yaw output
function [roll, pitch, yaw] = quat2eul_custom(w, x, y, z)
% 输入: w, x, y, z 四元数
% 输出: roll, pitch, yaw (ZYX顺序，单位：弧度)

q = [w, x, y, z];

% 计算欧拉角 (ZYX顺序)
yaw = atan2(2*(w*z + x*y), 1 - 2*(y^2 + z^2));
pitch = asin(2*(w*y - z*x));
roll = atan2(2*(w*x + y*z), 1 - 2*(x^2 + y^2));
end

== matlab function softdrone_pid/Control System/AttitudeControl/MATLAB Function1 ==
  data: imu_roll_gyro input; gyro_data_rotated output; imu_pitch_gyro input; imu_yaw_gyro input
function gyro_data_rotated = fcn(imu_roll_gyro, imu_pitch_gyro, imu_yaw_gyro)

% 定义角速度向量
gyro_data = [imu_roll_gyro; imu_pitch_gyro; imu_yaw_gyro];

% 定义绕 x 轴旋转 180 度的旋转矩阵
Rx_180 = [1  0  0;
          0 -1  0;
          0  0 -1];

% 应用旋转矩阵
gyro_data_rotated = Rx_180 * gyro_data;

== matlab function softdrone_pid/MATLAB Function12 ==
  data: u input; y output
function y = fcn(u)

RC_MIN = 341;
RC_MID = 1024;
RC_MAX = 1706;
DEADZONE = 20;

u = double(u);

if u > RC_MID + DEADZONE
    y = (u - RC_MID - DEADZONE) / ...
        (RC_MAX - RC_MID - DEADZONE);

elseif u < RC_MID - DEADZONE
    y = (u - RC_MID + DEADZONE) / ...
        (RC_MID - RC_MIN - DEADZONE);

else
    y = 0;
end

% 限幅
if y > 1
    y = 1;
elseif y < -1
    y = -1;
end

== matlab function softdrone_pid/MATLAB Function13 ==
  data: u input; y output
function y = fcn(u)

RC_MIN = 341;
RC_MID = 1024;
RC_MAX = 1706;
DEADZONE = 20;

u = double(u);

if u > RC_MID + DEADZONE
    y = (u - RC_MID - DEADZONE) / ...
        (RC_MAX - RC_MID - DEADZONE);

elseif u < RC_MID - DEADZONE
    y = (u - RC_MID + DEADZONE) / ...
        (RC_MID - RC_MIN - DEADZONE);

else
    y = 0;
end

% 限幅
if y > 1
    y = 1;
elseif y < -1
    y = -1;
end

== matlab function softdrone_pid/MATLAB Function14 ==
  data: u input; y output
function y = fcn(u)

RC_MIN = 341;
RC_MID = 1024;
RC_MAX = 1706;
DEADZONE = 20;

u = double(u);

if u > RC_MID + DEADZONE
    y = (u - RC_MID - DEADZONE) / ...
        (RC_MAX - RC_MID - DEADZONE);

elseif u < RC_MID - DEADZONE
    y = (u - RC_MID + DEADZONE) / ...
        (RC_MID - RC_MIN - DEADZONE);

else
    y = 0;
end

% 限幅
if y > 1
    y = 1;
elseif y < -1
    y = -1;
end

== matlab function softdrone_pid/MATLAB Function15 ==
  data: u input; y output
function y = fcn(u)

RC_MIN = 341;
RC_MID = 1024;
RC_MAX = 1706;
DEADZONE = 20;

u = double(u);

if u > RC_MID + DEADZONE
    y = (u - RC_MID - DEADZONE) / ...
        (RC_MAX - RC_MID - DEADZONE);

elseif u < RC_MID - DEADZONE
    y = (u - RC_MID + DEADZONE) / ...
        (RC_MID - RC_MIN - DEADZONE);

else
    y = 0;
end

% 限幅
if y > 1
    y = 1;
elseif y < -1
    y = -1;
end

== matlab function softdrone_pid/Control System/InputConditioning/f1 ==
  data: in input; y output; hover input
function y = thr_curve(in, hover)
%Function description:
%  throttle curve. When the throttle is in the middle position, the output
%  is hovering throttle value.
%Input:
%  in: normalized throttle, range from 0 to 1
%  hover: hovering throttle value
%Output:
%  y: processed throttle value
if in < 0.5
	y=2 * in * hover;
else
	y=hover + 2 * (in - 0.5) * (1.0 - hover);
end

== matlab function softdrone_pid/Control System/InputConditioning/deadzone2 ==
  data: u input; y output
function y = fcn(u)
%Function description:
%  Control the range of the remote control input from RCMin to RCMax, and
%  set a dead zone with a dead zone size of ±deadZone. The output y is
%  normalized to 0~1.You can get the RC calibration parameters in QGC.
RCMin = 1100;
RCMax = 1900;
RCMid = (RCMin + RCMax)/2;
deadZoneRate = 0.05;
deadZone = deadZoneRate*(RCMax - RCMin);
k = 1/(RCMax - RCMid - deadZone);
% saturation
if(u < RCMin)
    u = RCMin;
elseif(u > RCMax)
    u = RCMax;
end
%dead zone and normalize
 if(u > RCMid + deadZone)
    y = (u-RCMid - deadZone)*k;
 elseif(u < RCMid - deadZone)
     y = (u - RCMid + deadZone)*k;
 else
     y = 0;
 end

 end

== matlab function softdrone_pid/Control System/InputConditioning/deadzone3 ==
  data: u input; y output
function y = fcn(u)
%Function description:
%  Control the range of the remote control input from RCMin to RCMax, and
%  set a dead zone with a dead zone size of ±deadZone. The output y is
%  normalized to 0~1.You can get the RC calibration parameters in QGC.
RCMin = 1100;
RCMax = 1900;
RCMid = (RCMin + RCMax)/2;
deadZoneRate = 0.05;
deadZone = deadZoneRate*(RCMax - RCMin);
k = 1/(RCMax - RCMid - deadZone);
% saturation
if(u < RCMin)
    u = RCMin;
elseif(u > RCMax)
    u = RCMax;
end
%dead zone and normalize
 if(u > RCMid + deadZone)
    y = (u-RCMid - deadZone)*k;
 elseif(u < RCMid - deadZone)
     y = (u - RCMid + deadZone)*k;
 else
     y = 0;
 end

 end

== matlab function softdrone_pid/Control System/InputConditioning/deadzone4 ==
  data: u input; y output
function y = fcn(u)
%Function description:
%  Control the range of the remote control input from RCMin to RCMax, and
%  set a dead zone with a dead zone size of ±deadZone. The output y is
%  normalized to 0~1.You can get the RC calibration parameters in QGC.
RCMin = 1100;
RCMax = 1900;
RCMid = (RCMin + RCMax)/2;
deadZoneRate = 0.05;
deadZone = deadZoneRate*(RCMax - RCMin);
k = 1/(RCMax - RCMid - deadZone);
% saturation
if(u < RCMin)
    u = RCMin;
elseif(u > RCMax)
    u = RCMax;
end
%dead zone and normalize
 if(u > RCMid + deadZone)
    y = (u-RCMid - deadZone)*k;
 elseif(u < RCMid - deadZone)
     y = (u - RCMid + deadZone)*k;
 else
     y = 0;
 end

 end

== matlab function softdrone_pid/MATLAB Function ==
  data: imu_roll input; roll output; pitch output; yaw output; imu_pitch input; imu_yaw input
function [roll, pitch, yaw] = fcn(imu_roll, imu_pitch, imu_yaw)

roll = imu_roll;
yaw = imu_yaw;
pitch = imu_pitch;

== matlab function softdrone_pid/MATLAB Function1 ==
  data: imu_roll_gyro input; gyro_data_rotated output; imu_pitch_gyro input; imu_yaw_gyro input
function gyro_data_rotated = fcn(imu_roll_gyro, imu_pitch_gyro, imu_yaw_gyro)

% 定义角速度向量
gyro_data = [imu_roll_gyro; imu_pitch_gyro; imu_yaw_gyro];

% 定义绕 x 轴旋转 180 度的旋转矩阵
xy_flip_matrix = [1  0  0;
                  0 -1  0;
                  0  0 -1];

% 应用旋转矩阵
gyro_data_rotated = xy_flip_matrix* gyro_data;

== matlab function softdrone_pid/Subsystem4/MATLAB Function ==
  data: u input; y output
function y = fcn(u)

if u == 1
    y=2000;
elseif u == 3
    y=1500;
else
    y=1000;
end

== matlab function softdrone_pid/MATLAB Function2 ==
  data: u input; y output
function y = fcn(u)
% Onboard PWM output
% Input : PWM pulse width in us
% Output: uint16, limited to 1000~2000 us

u = double(u);

if u < 1000
    u = 1000;
elseif u > 2000
    u = 2000;
end

y = uint16(round(u));
end

== matlab function softdrone_pid/MATLAB Function3 ==
  data: u input; y output
function y = fcn(u)
% Onboard PWM output
% Input : PWM pulse width in us
% Output: uint16, limited to 1000~2000 us

u = double(u);

if u < 1000
    u = 1000;
elseif u > 2000
    u = 2000;
end

y = uint16(round(u));
end

== matlab function softdrone_pid/MATLAB Function4 ==
  data: u input; y output
function y = fcn(u)
% Onboard PWM output
% Input : PWM pulse width in us
% Output: uint16, limited to 1000~2000 us

u = double(u);

if u < 1000
    u = 1000;
elseif u > 2000
    u = 2000;
end

y = uint16(round(u));
end

== matlab function softdrone_pid/Control System/AttitudeControl/Eurle2quat ==
  data: roll input; quaternion output; pitch input; yaw input
function quaternion = fcn(roll, pitch, yaw)

eul = [yaw, pitch, roll];
quaternion = eul2quat(eul);
